simulink model "r2_b16a4x64f"  (R2012b)
(part 3 of 227)

  latch0/6(feng_chk_err_reg) -> status0/6(out_feng_chk_err)
  latch0/14(pack_err_reg) -> status0/14(out_pack_err)
  latch0/10(rx_bad_pkt_reg) -> status0/10(out_rx_bad_pkt)
  latch0/7(adc_over_reg) -> status0/7(out_adc_over)
  latch0/9(vacc_err_reg) -> status0/9(out_vacc_err)
  latch0/4(fft_err_reg) -> status0/4(out_fft_err)
  latch0/11(rx_bad_frame_reg) -> status0/11(out_rx_bad_frame)
  latch0/5(feng_qdr_err_reg) -> status0/5(out_feng_qdr_err)
  latch0/8(noise_diode_en_reg) -> status0/8(out_noise_diode_en)
  latch0/13(xeng_bad_dat_reg) -> status0/13(out_xeng_bad_dat)
  latch0/17(data_bad) -> [data_in_bad0]
  latch0/18(error) -> [err0]
  [gbe_up0] -> Inverter5/1
  [clr_status] -> latch0/1(reset)
  [pack_err0] -> latch0/15(pack_err)
  [pre_rx_dest_err0] -> latch0/3(rx_dest_err)
  [pre_feng_rx_err0] -> latch0/4(feng_rx_err)
  [pre_ndiode_en0] -> latch0/9(noise_diode_en)
  [pre_adc_err0] -> latch0/8(adc_over)
  [vacc_err0] -> latch0/10(vacc_err)
  [pre_spead_err0] -> latch0/11(rx_bad_pkt)
  [pre_feng_chk_err0] -> latch0/7(feng_chk_err)
  [gbe_rx_bad0] -> latch0/12(rx_bad_frame)
  [pre_feng_qdr_err0] -> latch0/6(feng_qdr_err)
  [gbe_tx_over0] -> latch0/13(tx_over)
  [pre_fft_err0] -> latch0/5(fft_err)
  [reord_recverr0] -> latch0/14(xeng_bad_dat)
  Inverter5/1 -> latch0/2(gbe_down)
  Inverter/1 -> latch0/16(rx)
  [accumulating0] -> latch0/17(tx)
  [reord_recverr0] -> Inverter/1
  [gbe_up1] -> Inverter7/1
  [clr_status] -> latch3/1(reset)
  [pack_err3] -> latch3/15(pack_err)
  [pre_rx_dest_err3] -> latch3/3(rx_dest_err)
  [pre_feng_rx_err3] -> latch3/4(feng_rx_err)
  [pre_ndiode_en3] -> latch3/9(noise_diode_en)
  [pre_adc_err3] -> latch3/8(adc_over)
  [vacc_err3] -> latch3/10(vacc_err)
  [pre_spead_err3] -> latch3/11(rx_bad_pkt)
  [pre_feng_chk_err3] -> latch3/7(feng_chk_err)
  [gbe_rx_bad1] -> latch3/12(rx_bad_frame)
  [pre_feng_qdr_err3] -> latch3/6(feng_qdr_err)
  [gbe_tx_over1] -> latch3/13(tx_over)
  [pre_fft_err3] -> latch3/5(fft_err)
  [reord_recverr3] -> latch3/14(xeng_bad_dat)
  Inverter7/1 -> latch3/2(gbe_down)
  Inverter6/1 -> latch3/16(rx)
  [accumulating3] -> latch3/17(tx)
  [reord_recverr3] -> Inverter6/1
  vacc_monitor7/1(pkt_cnt) -> packcnt_out3/1(out_reg)
  vacc_monitor7/2(error_cnt) -> packerr_3/1(out_reg)
  [cnt_rst] -> vacc_monitor7/1(cnt_rst)
  [pack_txeof3] -> vacc_monitor7/2(eof)
  [pack_err3] -> vacc_monitor7/3(error)
  [vacc_ld_stat3] -> Delay5/1(d)
  [err_output_of3] -> vacc_monitor11/5(outof)
  [err_parity3] -> vacc_monitor11/6(parity)
  [err_rst3] -> vacc_monitor11/4(rst)
  [err_input_of3] -> vacc_monitor11/3(inof)
  [err_calfail3] -> vacc_monitor11/2(cal)
  vacc_monitor11/1(cal_cnt) -> vacc_errors3/1(out_calfail)
  vacc_monitor11/2(inof_cnt) -> vacc_errors3/2(out_inputof)
  vacc_monitor11/3(rst_cnt) -> vacc_errors3/3(out_rst)
  vacc_monitor11/4(outof_cnt) -> vacc_errors3/4(out_outputof)
  vacc_monitor11/5(parity_cnt) -> vacc_errors3/5(out_parity)
  [vacc_err_flags3] -> bus_expand4/1(bus_in)
  miss_cnt3/3(recv_ctr) -> reordcnt_recv3/1(out_reg)
  miss_cnt3/1(spectr_cnt) -> reordcnt_spec3/1(out_reg)
  miss_cnt3/2(last_missed_ant) -> reord_missant3/1(out_reg)
  miss_cnt3/4(recv_errctr) -> reorderr_recv3/1(out_reg)
  miss_cnt3/5(timeout_errctr) -> reorderr_timeout3/1(out_reg)
  miss_cnt3/6(pktdisc_errctr) -> reorderr_disc3/1(out_reg)
  [flags_error0] -> Logical/1
  [flags_error1] -> Logical/2
  [flags_error2] -> Logical/3
  [flags_error3] -> Logical/4
  [flags_warning0] -> Logical1/1
  [flags_warning1] -> Logical1/2
  [flags_warning2] -> Logical1/3
  [flags_warning3] -> Logical1/4
  Logical/1 -> Slice/1
  Logical1/1 -> Slice1/1
  [cnt_rst] -> Delay3/2, Delay/2
  Delay/1 -> status/1(out_error)
  Delay3/1 -> status/2(out_warning)
  Slice/1 -> Delay/3, Delay/1
  Slice1/1 -> Delay3/3, Delay3/1
  Delay4/1(q) -> bus_expand5/1(bus_in)
  gapsize/1(in_gap_size) -> Register/1, Relational/2, Delay1/1
  Delay1/1 -> Relational/1
  Relational/1 -> Register/2
  Register/1 -> pipeline24/1(d), pipeline23/1(d), pipeline14/1(d), pipeline10/1(d)
  Delay5/1(q) -> bus_expand8/1(bus_in)
  [pack_ready0] -> vacc_monitor1/3(ready)
  [pack_txeof0] -> vacc_monitor1/4(eof)
  vacc_monitor1/2(ready_cnt) -> vaccout0/1(out_ready_cnt)
  vacc_monitor1/1(acc_cnt) -> vacccnt0/1(out_reg)
  vacc_monitor1/4(error_cnt) -> vaccerr0/1(out_reg)
  vacc_monitor1/3(eof_cnt) -> vaccout0/2(out_eof_cnt)
  vacc_monitor10/2(ready_cnt) -> vaccout1/1(out_ready_cnt)
  vacc_monitor10/1(acc_cnt) -> vacccnt1/1(out_reg)
  vacc_monitor10/4(error_cnt) -> vaccerr1/1(out_reg)
  vacc_monitor10/3(eof_cnt) -> vaccout1/2(out_eof_cnt)
  [vacc_err1] -> vacc_monitor10/5(error)
  [pack_txeof1] -> vacc_monitor10/4(eof)
  [pack_ready1] -> vacc_monitor10/3(ready)
  [vacc_newacc1] -> vacc_monitor10/2(new_acc)
  [cnt_rst] -> vacc_monitor10/1(cnt_rst), vacc_monitor9/1(cnt_rst)
  bus_expand7/1(msb_out2) -> vacc_ld_status2/1(out_armcnt)
  bus_expand7/2(lsb_out1) -> vacc_ld_status2/2(out_ldcnt)
  vacc_monitor4/1(acc_cnt) -> vacccnt2/1(out_reg)
  Delay39/1(q) -> bus_expand7/1(bus_in)
  [vacc_err2] -> vacc_monitor4/5(error)
  [pack_ready2] -> vacc_monitor4/3(ready)
  [pack_txeof2] -> vacc_monitor4/4(eof)
  [vacc_newacc2] -> vacc_monitor4/2(new_acc)
  bus_expand8/1(msb_out2) -> vacc_ld_status3/1(out_armcnt)
  bus_expand8/2(lsb_out1) -> vacc_ld_status3/2(out_ldcnt)
  vacc_monitor12/2(ready_cnt) -> vaccout3/1(out_ready_cnt)
  vacc_monitor12/1(acc_cnt) -> vacccnt3/1(out_reg)
  vacc_monitor12/4(error_cnt) -> vaccerr3/1(out_reg)
  vacc_monitor12/3(eof_cnt) -> vaccout3/2(out_eof_cnt)
  [pack_ready2] -> vacc_monitor12/3(ready)
  [pack_txeof2] -> vacc_monitor12/4(eof)
  [vacc_err3] -> vacc_monitor12/5(error)
  [cnt_rst] -> vacc_monitor12/1(cnt_rst), vacc_monitor11/1(cnt_rst)
  [vacc_newacc3] -> vacc_monitor12/2(new_acc)
  vacc_monitor4/4(error_cnt) -> vaccerr2/1(out_reg)
  vacc_monitor4/3(eof_cnt) -> vaccout2/2(out_eof_cnt)
  vacc_monitor4/2(ready_cnt) -> vaccout2/1(out_ready_cnt)
  [flush0] -> latch0/18(flush)
  latch0/19(flush_reg) -> status0/17(out_flushed)
  [flush0] -> latch1/18(flush)
  latch1/15(rx_reg) -> status1/15(out_rxing_data)
  latch1/6(feng_chk_err_reg) -> status1/6(out_feng_chk_err)
  latch1/1(gbe_down_reg) -> status1/1(out_gbe_down)
  latch1/12(tx_over_reg) -> status1/12(out_tx_over)
  latch1/13(xeng_bad_dat_reg) -> status1/13(out_xeng_bad_dat)
  latch1/10(rx_bad_pkt_reg) -> status1/10(out_rx_bad_pkt)
  latch1/9(vacc_err_reg) -> status1/9(out_vacc_err)
  latch1/2(rx_dest_err_reg) -> status1/2(out_rx_dest_err)
  latch1/3(feng_rx_err_reg) -> status1/3(out_feng_rx_err)
  latch1/11(rx_bad_frame_reg) -> status1/11(out_rx_bad_frame)
  latch1/7(adc_over_reg) -> status1/7(out_adc_over)
  latch1/5(feng_qdr_err_reg) -> status1/5(out_feng_qdr_err)
  latch1/14(pack_err_reg) -> status1/14(out_pack_err)
  latch1/16(tx_reg) -> status1/16(out_txing_data)
  latch1/8(noise_diode_en_reg) -> status1/8(out_noise_diode_en)
  latch1/4(fft_err_reg) -> status1/4(out_fft_err)
  latch1/17(data_bad) -> [data_in_bad1]
  latch1/18(error) -> [err1]
  latch1/19(flush_reg) -> status1/17(out_flushed)
  [flush1] -> latch2/18(flush)
  [flush1] -> latch3/18(flush)
  latch2/14(pack_err_reg) -> status2/14(out_pack_err)
  latch2/7(adc_over_reg) -> status2/7(out_adc_over)
  latch2/10(rx_bad_pkt_reg) -> status2/10(out_rx_bad_pkt)
  latch2/1(gbe_down_reg) -> status2/1(out_gbe_down)
  latch2/16(tx_reg) -> status2/16(out_txing_data)
  latch2/6(feng_chk_err_reg) -> status2/6(out_feng_chk_err)
  latch2/12(tx_over_reg) -> status2/12(out_tx_over)
  latch2/11(rx_bad_frame_reg) -> status2/11(out_rx_bad_frame)
  latch2/2(rx_dest_err_reg) -> status2/2(out_rx_dest_err)
  latch2/8(noise_diode_en_reg) -> status2/8(out_noise_diode_en)
  latch2/3(feng_rx_err_reg) -> status2/3(out_feng_rx_err)
  latch2/15(rx_reg) -> status2/15(out_rxing_data)
  latch2/5(feng_qdr_err_reg) -> status2/5(out_feng_qdr_err)
  latch2/4(fft_err_reg) -> status2/4(out_fft_err)
  latch2/9(vacc_err_reg) -> status2/9(out_vacc_err)
  latch2/13(xeng_bad_dat_reg) -> status2/13(out_xeng_bad_dat)
  latch2/17(data_bad) -> [data_in_bad2]
  latch2/18(error) -> [err2]
  latch2/19(flush_reg) -> status2/17(out_flushed)
  latch3/6(feng_chk_err_reg) -> status3/6(out_feng_chk_err)
  latch3/1(gbe_down_reg) -> status3/1(out_gbe_down)
  latch3/12(tx_over_reg) -> status3/12(out_tx_over)
  latch3/13(xeng_bad_dat_reg) -> status3/13(out_xeng_bad_dat)
  latch3/15(rx_reg) -> status3/15(out_rxing_data)
  latch3/7(adc_over_reg) -> status3/7(out_adc_over)
  latch3/8(noise_diode_en_reg) -> status3/8(out_noise_diode_en)
  latch3/11(rx_bad_frame_reg) -> status3/11(out_rx_bad_frame)
  latch3/16(tx_reg) -> status3/16(out_txing_data)
  latch3/10(rx_bad_pkt_reg) -> status3/10(out_rx_bad_pkt)
  latch3/9(vacc_err_reg) -> status3/9(out_vacc_err)
  latch3/3(feng_rx_err_reg) -> status3/3(out_feng_rx_err)
  latch3/14(pack_err_reg) -> status3/14(out_pack_err)
  latch3/4(fft_err_reg) -> status3/4(out_fft_err)
  latch3/5(feng_qdr_err_reg) -> status3/5(out_feng_qdr_err)
  latch3/2(rx_dest_err_reg) -> status3/2(out_rx_dest_err)
  latch3/17(data_bad) -> [data_in_bad3]
  latch3/19(flush_reg) -> status3/17(out_flushed)
  latch3/18(error) -> [err3]
  bus_expand2/1(msb_out5) -> [err_parity0]
  bus_expand2/2(out4) -> [err_output_of0]
  bus_expand2/3(out3) -> [err_rst0]
  bus_expand2/4(out2) -> [err_input_of0]
  bus_expand2/5(lsb_out1) -> [err_calfail0]
  bus_expand1/1(msb_out5) -> [err_parity1]
  bus_expand1/2(out4) -> [err_output_of1]
  bus_expand1/3(out3) -> [err_rst1]
  bus_expand1/4(out2) -> [err_input_of1]
  bus_expand1/5(lsb_out1) -> [err_calfail1]
  bus_expand9/1(msb_out5) -> [err_parity2]
  bus_expand9/2(out4) -> [err_output_of2]
  bus_expand9/3(out3) -> [err_rst2]
  bus_expand9/4(out2) -> [err_input_of2]
  bus_expand9/5(lsb_out1) -> [err_calfail2]
  bus_expand4/1(msb_out5) -> [err_parity3]
  bus_expand4/2(out4) -> [err_output_of3]
  bus_expand4/3(out3) -> [err_rst3]
  bus_expand4/4(out2) -> [err_input_of3]
  bus_expand4/5(lsb_out1) -> [err_calfail3]
  [pre_rx_dest_err0] -> Subsystem5/5(dest_err)
  Subsystem5/3(desterr_cnt) -> dest_err_cnt0/1(out_reg)
  [spead_error1] -> Subsystem2/4(flag)
  [spead_eof1] -> Subsystem2/3(eof)
  [spead_valid1] -> Subsystem2/2(we)
  Subsystem2/1(rx_cnt) -> rx_cnt1/1(out_reg)
  Subsystem2/2(err_cnt) -> rx_err_cnt1/1(out_reg)
  Subsystem2/3(desterr_cnt) -> dest_err_cnt1/1(out_reg)
  [pre_rx_dest_err1] -> Subsystem2/5(dest_err)
  Constant4/1 -> gbe2/7(rx_ack)
  Constant5/1 -> gbe2/8(rx_overrun_ack)
  Constant6/1 -> gbe3/7(rx_ack)
  Constant3/1 -> gbe3/8(rx_overrun_ack)
  [gbe_debug_rst] -> gbe2/9(debug_rst)
  [gbe_debug_rst] -> gbe3/9(debug_rst)
  [gbe_rst] -> gbe2/1(rst)
  [gbe_txd2] -> gbe2/2(tx_data)
  [gbe_txvld2] -> gbe2/3(tx_valid)
  [gbe_txeof2] -> gbe2/6(tx_end_of_frame)
  [gbe_rst] -> gbe3/1(rst)
  [gbe_txd3] -> gbe3/2(tx_data)
  [gbe_txvld3] -> gbe3/3(tx_valid)
  [gbe_txeof3] -> gbe3/6(tx_end_of_frame)
  Constant7/1 -> [gbe_txd2]
  Constant10/1 -> [gbe_txvld2]
  Constant11/1 -> [gbe_txeof2]
  Constant15/1 -> [gbe_txd3]
  Constant12/1 -> [gbe_txvld3]
  Constant14/1 -> [gbe_txeof3]
  [gbe_rxvld2] -> Delay41/1(d)
  [gbe_rxdata2] -> Delay40/1(d)
  [gbe_rxeof2] -> Delay42/1(d)
  Delay40/1(q) -> spead_unpack2/1(pkt_data)
  Delay41/1(q) -> spead_unpack2/2(pkt_valid)
  Delay42/1(q) -> spead_unpack2/3(pkt_eof)
  [gbe_rxvld3] -> Delay44/1(d)
  [gbe_rxdata3] -> Delay43/1(d)
  [gbe_rxeof3] -> Delay45/1(d)
  Delay43/1(q) -> spead_unpack3/1(pkt_data)
  Delay44/1(q) -> spead_unpack3/2(pkt_valid)
  Delay45/1(q) -> spead_unpack3/3(pkt_eof)
  [cnt_rst] -> Subsystem1/1(rst)
  [spead_error2] -> Subsystem1/4(flag)
  [spead_eof2] -> Subsystem1/3(eof)
  [spead_valid2] -> Subsystem1/2(we)
  Subsystem1/1(rx_cnt) -> rx_cnt2/1(out_reg)
  Subsystem1/2(err_cnt) -> rx_err_cnt2/1(out_reg)
  Subsystem1/3(desterr_cnt) -> dest_err_cnt2/1(out_reg)
  [pre_rx_dest_err2] -> Subsystem1/5(dest_err)
  [cnt_rst] -> Subsystem3/1(rst)
  [spead_error3] -> Subsystem3/4(flag)
  [spead_eof3] -> Subsystem3/3(eof)
  [spead_valid3] -> Subsystem3/2(we)
  Subsystem3/1(rx_cnt) -> rx_cnt3/1(out_reg)
  Subsystem3/2(err_cnt) -> rx_err_cnt3/1(out_reg)
  Subsystem3/3(desterr_cnt) -> dest_err_cnt3/1(out_reg)
  [pre_rx_dest_err3] -> Subsystem3/5(dest_err)
  bf_config/1(in_data_id) -> pipeline26/1(d)
  bf_config/2(in_time_id) -> pipeline27/1(d)
  bf_control/2(in_stream) -> pipeline29/1(d)
  bf_control/3(in_antenna) -> pipeline30/1(d)
  bf_control/1(in_beng) -> pipeline28/1(d)
  pipeline26/1(q) -> [bf_data_id]
  pipeline27/1(q) -> [bf_time_id]
  pipeline28/1(q) -> [bf_beng]
  pipeline29/1(q) -> [bf_stream]
  pipeline30/1(q) -> [bf_antenna]
  pipeline53/1(q) -> [bf_value_filt]
  pipeline54/1(q) -> [bf_value_dupl]
  pipeline55/1(q) -> [bf_value_bw]
  pipeline56/1(q) -> [bf_value_quant]
  bf_value_in0/1(in_dupl) -> pipeline54/1(d)
  bf_value_in1/1(in_quant) -> pipeline56/1(d)
  bf_value_in1/2(in_filt) -> pipeline53/1(d)
  bf_value_ctrl/1(in_dupl) -> pipeline32/1(d)
  bf_value_ctrl/3(in_quant) -> pipeline34/1(d)
  pipeline32/1(q) -> edge_detect6/1
  pipeline33/1(q) -> edge_detect7/1
  pipeline34/1(q) -> edge_detect8/1
  pipeline57/1(q) -> edge_detect9/1
  bf_value_ctrl/2(in_bw) -> pipeline33/1(d)
  bf_value_ctrl/4(in_filt) -> pipeline57/1(d)
  bf_value_in0/2(in_bw) -> pipeline55/1(d)
  [bfout_valbw0] -> Delay27/1(d)
  [bfout_valquant0] -> Delay30/1(d)
  [bfout_valfilt0] -> Delay31/1(d)
  [bfout_valbw1] -> Delay26/1(d)
  [bfout_valbw2] -> Delay28/1(d)
  [bfout_valbw3] -> Delay32/1(d)
  [bfout_valquant1] -> Delay33/1(d)
  [bfout_valquant2] -> Delay35/1(d)
  [bfout_valquant3] -> Delay36/1(d)
  [bfout_valfilt1] -> Delay37/1(d)
  [bfout_valfilt2] -> Delay38/1(d)
  [bfout_valfilt3] -> Delay46/1(d)
  Delay27/1(q) -> bf_valout_bw0/1(out_bw0)
  Delay26/1(q) -> bf_valout_bw0/2(out_bw1)
  Delay32/1(q) -> bf_valout_bw1/2(out_bw3)
  Delay28/1(q) -> bf_valout_bw1/1(out_bw2)
  Delay30/1(q) -> bf_valout_quant0/1(out_quant0)
  Delay33/1(q) -> bf_valout_quant0/2(out_quant1)
  Delay36/1(q) -> bf_valout_quant1/2(out_quant3)
  Delay35/1(q) -> bf_valout_quant1/1(out_quant2)
  Delay37/1(q) -> bf_valout_filt/2(out_filt1)
  Delay38/1(q) -> bf_valout_filt/3(out_filt2)
  Delay46/1(q) -> bf_valout_filt/4(out_filt3)
  Delay31/1(q) -> bf_valout_filt/1(out_filt0)
  edge_detect6/1 -> [bf_valctrl_dupl]
  edge_detect7/1 -> [bf_valctrl_bw]
  edge_detect8/1 -> [bf_valctrl_quant]
  edge_detect9/1 -> [bf_valctrl_filt]
  Concat5/1 -> gbe_mux_bus0/1(di)
  [pack_txd1] -> Concat5/2
  [pack_txd0] -> Concat5/1
  Concat6/1 -> gbe_mux_bus0/2(validi)
  Concat7/1 -> gbe_mux_bus0/3(eofi)
  gbe_mux_bus0/5(start) -> Delay12/1, bus_expand/1(bus_in)
  Concat9/1 -> gbe_mux_bus0/4(drdy)
  Constant26/1 -> gbe_mux_bus0/5(transmit)
  gbe_mux_bus0/2(do) -> Delay13/1
  gbe_mux_bus0/3(valido) -> Delay14/1
  gbe_mux_bus0/4(eofo) -> Delay15/1
  gbe_mux_bus0/6(flush) -> [flush0]
  [bf0s_d0] -> Concat5/3
  [bf1s_d0] -> Concat5/4
  [pack_txvld0] -> Concat6/1
  [pack_txvld1] -> Concat6/2
  [bf0s_en0] -> Concat6/3
  [bf1s_en0] -> Concat6/4
  [bf0s_eof0] -> Concat7/3
  [bf1s_eof0] -> Concat7/4
  [pack_txeof0] -> Concat7/1
  [pack_txeof1] -> Concat7/2
  [bf0s_pkt_ready0] -> Concat9/3
  [bf1s_pkt_ready0] -> Concat9/4
  [pack_ready1] -> Concat9/2
  [pack_ready0] -> Concat9/1
  [bf0s_d1] -> Concat5/5
  [bf1s_d1] -> Concat5/6
  [bf0s_en1] -> Concat6/5
  [bf1s_en1] -> Concat6/6
  [bf0s_eof1] -> Concat7/5
  [bf1s_eof1] -> Concat7/6
  [bf0s_pkt_ready1] -> Concat9/5
  [bf1s_pkt_ready1] -> Concat9/6
  bus_expand/1(msb_out6) -> [go0]
  bus_expand/2(out5) -> [go1]
  bus_expand/3(out4) -> [bf0_tx_pkt0]
  bus_expand/4(out3) -> [bf1_tx_pkt0]
  bus_expand/5(out2) -> [bf0_tx_pkt1]
  bus_expand/6(lsb_out1) -> [bf1_tx_pkt1]
  Concat1/1 -> gbe_mux_bus/1(di)
  Concat2/1 -> gbe_mux_bus/2(validi)
  Concat3/1 -> gbe_mux_bus/3(eofi)
  gbe_mux_bus/5(start) -> bus_expand3/1(bus_in)
  Concat4/1 -> gbe_mux_bus/4(drdy)
  Constant1/1 -> gbe_mux_bus/5(transmit)
  gbe_mux_bus/2(do) -> Delay24/1
  gbe_mux_bus/4(eofo) -> Delay22/1
  gbe_mux_bus/6(flush) -> [flush1]
  gbe_mux_bus/3(valido) -> Delay23/1
  [pack_txd2] -> Concat1/1
  [pack_txd3] -> Concat1/2
  [pack_txvld2] -> Concat2/1
  [pack_txvld3] -> Concat2/2
  [pack_txeof2] -> Concat3/1
  [pack_txeof3] -> Concat3/2
  [pack_ready2] -> Concat4/1
  [pack_ready3] -> Concat4/2
  bus_expand3/1(msb_out6) -> [go2]
  bus_expand3/2(out5) -> [go3]
  [bf0s_d2] -> Concat1/3
  [bf1s_d2] -> Concat1/4
  [bf0s_d3] -> Concat1/5
  [bf1s_d3] -> Concat1/6
  [bf0s_en2] -> Concat2/3
  [bf1s_en2] -> Concat2/4
  [bf0s_en3] -> Concat2/5
  [bf1s_en3] -> Concat2/6
  [bf0s_eof2] -> Concat3/3
  [bf1s_eof2] -> Concat3/4
  [bf0s_eof3] -> Concat3/5
  [bf1s_eof3] -> Concat3/6
  [bf0s_pkt_ready2] -> Concat4/3
  [bf1s_pkt_ready2] -> Concat4/4
  [bf0s_pkt_ready3] -> Concat4/5
  [bf1s_pkt_ready3] -> Concat4/6
  bus_expand3/3(out4) -> [bf0_tx_pkt2]
  bus_expand3/4(out3) -> [bf1_tx_pkt2]
  bus_expand3/5(out2) -> [bf0_tx_pkt3]
  bus_expand3/6(lsb_out1) -> [bf1_tx_pkt3]
  Delay13/1 -> [gbe_txd0]
  Delay14/1 -> [gbe_txvld0]
  Delay15/1 -> [gbe_txeof0]
  gbe_mux_bus0/1(input) -> Mux2/1, Delay11/1, Mux1/1
  AddSub7/1 -> Mux1/5
  AddSub4/1 -> Mux1/4
  [bf0_txport] -> Mux2/6, Mux2/4
  [bf1_txport] -> Mux2/7, Mux2/5
  [gbe_txport] -> Mux2/3, Mux2/2
  Mux2/1 -> [gbe_txport0]
  Delay22/1 -> [gbe_txeof1]
  Delay23/1 -> [gbe_txvld1]
  Delay24/1 -> [gbe_txd1]
  gbe_mux_bus/1(input) -> Mux3/1, Mux4/1
  AddSub13/1 -> Mux3/5
  AddSub10/1 -> Mux3/4
  [bf0_txport] -> Mux4/4, Mux4/6
  [bf1_txport] -> Mux4/7, Mux4/5
  [gbe_txport] -> Mux4/2, Mux4/3
  Mux3/1 -> [gbe_txip1]
  Mux4/1 -> [gbe_txport1]
  Delay11/1 -> [gbe_ipsel0]
  Delay12/1 -> [gbe_txstart0]
  Mux1/1 -> [gbe_txip0]
  Constant18/1 -> gbe3/4(tx_dest_ip)
  Constant19/1 -> gbe3/5(tx_dest_port)
  Constant16/1 -> gbe2/4(tx_dest_ip)
  Constant17/1 -> gbe2/5(tx_dest_port)
  pipeline59/1(q) -> [bf_tvgsel]
  bf_config/3(in_tvg_sel) -> pipeline59/1(d)
  pipeline60/1(q) -> [bf_snap_arm]
  pipeline61/1(q) -> [bf_snap_trig]
  bf_config/4(in_snap_arm) -> pipeline60/1(d)
  bf_config/5(in_snap_trig) -> pipeline61/1(d)
  [bfout_sync0] -> Delay53/1(d)
  [bf_snap_arm] -> Logical4/1
  Delay53/1(q) -> Logical4/2
  Logical4/1 -> Logical5/1
  [bf_snap_trig] -> edge_detect10/1
  edge_detect10/1 -> Logical5/2
  Logical5/1 -> bfsnap_out/6(trig)
  [bfout_sync0] -> Delay54/1(d)
  [bfout_den0] -> slice1/1
  Delay56/1(q) -> bfsnap_out/3(in_d32)
  [bfout_d0] -> Delay56/1(d)
  Delay57/1(q) -> slice5/1
  [bfout_time0] -> Delay57/1(d)
  Delay54/1(q) -> bfsnap_out/1(in_sync)
  Delay55/1(q) -> bfsnap_out/2(in_en), bfsnap_out/5(we)
  slice5/1 -> bfsnap_out/4(in_time27)
  slice1/1 -> Delay55/1(d)
  vacctvg_control/1(in_sync_sel) -> pipeline65/1(d)
  vacctvg_control/2(in_valid_sel) -> pipeline62/1(d)
  vacctvg_control/3(in_data_sel) -> pipeline66/1(d)
  vacctvg_control/4(in_reset) -> pipeline64/1(d)
  vacctvg_control/5(in_ctr_en) -> pipeline69/1(d)
  vacctvg_control/6(in_vector_en) -> pipeline67/1(d)
  vacctvg_control/7(in_pulse_en) -> pipeline70/1(d)
  pipeline65/1(q) -> [vacctvg_sync_sel]
  pipeline62/1(q) -> [vacctvg_valid_sel]
  pipeline64/1(q) -> [vacctvg_reset]
  pipeline66/1(q) -> [vacctvg_data_sel]
  pipeline67/1(q) -> [vacctvg_vector_en]
  pipeline69/1(q) -> [vacctvg_ctr_en]
  pipeline70/1(q) -> [vacctvg_pulse_en]
  pipeline68/1(q) -> [vacctvg_vbs_rst0]
  vacctvg_control/8(in_vbs_rst0) -> pipeline68/1(d)
  pipeline71/1(q) -> [vacctvg_vbs_rst1]
  pipeline63/1(q) -> [vacctvg_vbs_rst2]
  pipeline72/1(q) -> [vacctvg_vbs_rst3]
  vacctvg_control/9(in_vbs_rst1) -> pipeline71/1(d)
  vacctvg_control/10(in_vbs_rst2) -> pipeline63/1(d)
  vacctvg_control/11(in_vbs_rst3) -> pipeline72/1(d)
  bf1_config/2(in_beam_id) -> pipeline58/1(d)
  bf1_config/1(in_rst) -> pipeline45/1(d)
  pipeline45/1(q) -> [bf1_rst]
  pipeline58/1(q) -> Convert1/1
  bf1_config/3(in_port) -> pipeline43/1(d)
  pipeline43/1(q) -> [bf1_txport]
  pipeline44/1(q) -> [bf1_txen]
  bf1_config/4(in_txen) -> pipeline44/1(d)
  Convert1/1 -> [bf1_id]
  pipeline37/1(q) -> [bf1_n_partitions]
  bf0_config/2(in_beam_id) -> pipeline50/1(d)
  bf0_config/1(in_rst) -> pipeline38/1(d)
  pipeline38/1(q) -> [bf0_rst]
  pipeline50/1(q) -> Convert2/1
  bf0_config/3(in_port) -> pipeline35/1(d)
  pipeline35/1(q) -> [bf0_txport]
  pipeline36/1(q) -> [bf0_txen]
  bf0_config/4(in_txen) -> pipeline36/1(d)
  Convert2/1 -> [bf0_id]
  bf0_num_parts/1(in_n_partitions) -> pipeline31/1(d)
  pipeline31/1(q) -> [bf0_n_partitions]
  bf0_partitions/1(in_partition0_offset) -> pipeline39/1(d)
  bf0_partitions/2(in_partition1_offset) -> pipeline40/1(d)
  bf0_partitions/3(in_partition2_offset) -> pipeline41/1(d)
  bf0_partitions/4(in_partition3_offset) -> pipeline42/1(d)
  bf1_partitions/1(in_partition0_offset) -> pipeline46/1(d)
  bf1_partitions/2(in_partition1_offset) -> pipeline47/1(d)
  bf1_partitions/3(in_partition2_offset) -> pipeline48/1(d)
  bf1_partitions/4(in_partition3_offset) -> pipeline49/1(d)
  pipeline39/1(q) -> [bf0_partition_offset0]
  pipeline40/1(q) -> [bf0_partition_offset1]
  pipeline41/1(q) -> [bf0_partition_offset2]
  pipeline42/1(q) -> [bf0_partition_offset3]
  pipeline46/1(q) -> [bf1_partition_offset0]
  pipeline47/1(q) -> [bf1_partition_offset1]
  pipeline48/1(q) -> [bf1_partition_offset2]
  pipeline49/1(q) -> [bf1_partition_offset3]
  bf0_ip/1(in_ip) -> pipeline51/1(d)
  pipeline51/1(q) -> [bf0_txip]
  bf1_ip/1(in_ip) -> pipeline52/1(d)
  pipeline52/1(q) -> [bf1_txip]
  [cnt_rst] -> Subsystem/1(rst)
  [bf0s_eof0] -> Subsystem/2(of0)
  Subsystem/1(Out1) -> bf0_out_count/1(out_count0)
  [bf0s_eof2] -> Subsystem/4(of2)
  [bf0s_eof1] -> Subsystem/3(of1)
  [bf0s_eof3] -> Subsystem/5(of3)
  Subsystem/2(Out2) -> bf0_out_count/2(out_count1)
  Subsystem/3(Out3) -> bf0_out_count/3(out_count2)
  Subsystem/4(Out4) -> bf0_out_count/4(out_count3)
  [cnt_rst] -> Subsystem4/1(rst)
  [bf0s_of0] -> Subsystem4/2(of0)
  Subsystem4/1(Out1) -> bf0_of_count/1(out_count0)
  [bf0s_of2] -> Subsystem4/4(of2)
  [bf0s_of1] -> Subsystem4/3(of1)
  [bf0s_of3] -> Subsystem4/5(of3)
  Subsystem4/2(Out2) -> bf0_of_count/2(out_count1)
  Subsystem4/3(Out3) -> bf0_of_count/3(out_count2)
  Subsystem4/4(Out4) -> bf0_of_count/4(out_count3)
  [cnt_rst] -> Subsystem6/1(rst)
  [bf1s_eof0] -> Subsystem6/2(of0)
  Subsystem6/1(Out1) -> bf1_out_count/1(out_count0)
  [bf1s_eof2] -> Subsystem6/4(of2)
  [bf1s_eof1] -> Subsystem6/3(of1)
  [bf1s_eof3] -> Subsystem6/5(of3)
  Subsystem6/2(Out2) -> bf1_out_count/2(out_count1)
  Subsystem6/3(Out3) -> bf1_out_count/3(out_count2)
  Subsystem6/4(Out4) -> bf1_out_count/4(out_count3)
  [cnt_rst] -> Subsystem7/1(rst)
  [bf1s_of0] -> Subsystem7/2(of0)
  Subsystem7/1(Out1) -> bf1_of_count/1(out_count0)
  [bf1s_of2] -> Subsystem7/4(of2)
  [bf1s_of1] -> Subsystem7/3(of1)
  [bf1s_of3] -> Subsystem7/5(of3)
  Subsystem7/3(Out3) -> bf1_of_count/3(out_count2)
  Subsystem7/4(Out4) -> bf1_of_count/4(out_count3)
  Subsystem7/2(Out2) -> bf1_of_count/2(out_count1)
  bf1_num_parts/1(in_n_partitions) -> pipeline37/1(d)
  gbe0/1(led_up) -> [gbe_up0]
  gbe0/3(led_tx) -> Terminator1/1
  gbe0/2(led_rx) -> Terminator7/1
  gbe0/4(tx_afull) -> Terminator13/1
  gbe0/5(tx_overflow) -> [gbe_tx_over0]
  gbe0/6(rx_data) -> [gbe_rxdata0]
  gbe0/7(rx_valid) -> [gbe_rxvld0]
  gbe0/8(rx_source_ip) -> Terminator14/1
  gbe0/9(rx_source_port) -> Terminator15/1
  gbe0/10(rx_end_of_frame) -> [gbe_rxeof0]
  gbe0/11(rx_bad_frame) -> [gbe_rx_bad0]
  gbe0/12(rx_overrun) -> Terminator35/1
  gbe0/13(rx_dest_ip) -> Terminator36/1
  gbe0/14(rx_dest_port) -> Terminator45/1
  gbe1/1(led_up) -> [gbe_up1]
  gbe1/2(led_rx) -> Terminator47/1
  gbe1/3(led_tx) -> Terminator38/1
  gbe1/4(tx_afull) -> Terminator46/1
  gbe1/5(tx_overflow) -> [gbe_tx_over1]
  gbe1/6(rx_data) -> [gbe_rxdata1]
  gbe1/7(rx_valid) -> [gbe_rxvld1]
  gbe1/8(rx_source_ip) -> Terminator48/1
  gbe1/9(rx_source_port) -> Terminator49/1
  gbe1/10(rx_end_of_frame) -> [gbe_rxeof1]
  gbe1/11(rx_bad_frame) -> [gbe_rx_bad1]
  gbe1/12(rx_overrun) -> Terminator50/1
  gbe1/13(rx_dest_ip) -> Terminator51/1
  gbe1/14(rx_dest_port) -> Terminator52/1
  gbe2/1(led_up) -> [gbe_up2]
  gbe2/5(tx_overflow) -> [gbe_tx_over2]
  gbe2/6(rx_data) -> [gbe_rxdata2]
  gbe2/7(rx_valid) -> [gbe_rxvld2]
  gbe2/10(rx_end_of_frame) -> [gbe_rxeof2]
  gbe2/11(rx_bad_frame) -> [gbe_rx_bad2]
  gbe3/1(led_up) -> [gbe_up3]
  gbe3/5(tx_overflow) -> [gbe_tx_over3]
  gbe3/6(rx_data) -> [gbe_rxdata3]
  gbe3/7(rx_valid) -> [gbe_rxvld3]
  gbe3/10(rx_end_of_frame) -> [gbe_rxeof3]
  gbe3/11(rx_bad_frame) -> [gbe_rx_bad3]
  gbe2/12(rx_overrun) -> Terminator6/1
  gbe2/13(rx_dest_ip) -> Terminator8/1
  gbe2/14(rx_dest_port) -> Terminator9/1
  gbe2/2(led_rx) -> Terminator10/1
  gbe2/3(led_tx) -> Terminator12/1
  gbe2/4(tx_afull) -> Terminator16/1
  gbe2/8(rx_source_ip) -> Terminator20/1
  gbe2/9(rx_source_port) -> Terminator21/1
  gbe3/12(rx_overrun) -> Terminator22/1
  gbe3/13(rx_dest_ip) -> Terminator24/1
  gbe3/14(rx_dest_port) -> Terminator25/1
  gbe3/2(led_rx) -> Terminator26/1
  gbe3/3(led_tx) -> Terminator53/1
  gbe3/4(tx_afull) -> Terminator54/1
  gbe3/8(rx_source_ip) -> Terminator55/1
  gbe3/9(rx_source_port) -> Terminator56/1
  [gbe_txip] -> AddSub6/1
  AddSub6/1 -> Mux1/2
  AddSub1/1 -> Mux1/3
  [gbe_txip] -> AddSub1/1
  [id1] -> AddSub5/2, AddSub8/2, AddSub1/2
  [gbe_txip] -> AddSub2/1
  [id2] -> AddSub13/2, AddSub10/2, AddSub2/2
  [gbe_txip] -> AddSub3/1
  [id3] -> AddSub3/2, AddSub14/2, AddSub11/2
  AddSub3/1 -> Mux3/3
  AddSub2/1 -> Mux3/2
  spead_unpack0/10(hdr5_0x1600_DIR) -> [spead_hdr1_0]
  spead_unpack0/11(hdr6_0x4101_DIR) -> [spead_hdr2_0]
  spead_unpack0/12(hdr7_0x4103_DIR) -> [spead_hdr3_0]
  spead_unpack0/13(hdr8_0x0000_DIR) -> Terminator33/1
  spead_unpack0/14(hdr9_0x0000_DIR) -> Terminator19/1
  spead_unpack0/15(hdr10_0x0000_DIR) -> Terminator4/1
  spead_unpack0/16(hdr11_0x4300) -> Terminator31/1
  spead_unpack1/2(data64) -> [spead_data1]
  spead_unpack1/3(valid64) -> [spead_valid1]
  spead_unpack1/4(eof64) -> [spead_eof1]
  spead_unpack1/5(error) -> [spead_error1]
  spead_unpack1/6(hdr_heap_id) -> Terminator17/1
  spead_unpack1/7(hdr_heap_size) -> Terminator18/1
  spead_unpack1/8(hdr_heap_offset) -> [spead_heap_offset1]
  spead_unpack1/9(hdr_pkt_len) -> Terminator32/1
  spead_unpack1/10(hdr5_0x1600_DIR) -> [spead_hdr1_1]
  spead_unpack1/11(hdr6_0x4101_DIR) -> [spead_hdr2_1]
  spead_unpack1/12(hdr7_0x4103_DIR) -> [spead_hdr3_1]
  spead_unpack1/16(hdr11_0x4300) -> Terminator42/1
  spead_unpack1/15(hdr10_0x0000_DIR) -> Terminator58/1
  spead_unpack1/14(hdr9_0x0000_DIR) -> Terminator11/1
  spead_unpack1/13(hdr8_0x0000_DIR) -> Terminator57/1
  spead_unpack2/1(pkt_start) -> Terminator34/1
  spead_unpack2/2(data64) -> [spead_data2]
  spead_unpack2/3(valid64) -> [spead_valid2]
  spead_unpack2/4(eof64) -> [spead_eof2]
  spead_unpack2/5(error) -> [spead_error2]
  spead_unpack2/6(hdr_heap_id) -> Terminator29/1
  spead_unpack2/7(hdr_heap_size) -> Terminator30/1
  spead_unpack2/8(hdr_heap_offset) -> [spead_heap_offset2]
  spead_unpack2/9(hdr_pkt_len) -> Terminator27/1
  spead_unpack2/10(hdr5_0x1600_DIR) -> [spead_hdr1_2]
  spead_unpack2/11(hdr6_0x4101_DIR) -> [spead_hdr2_2]
  spead_unpack2/12(hdr7_0x4103_DIR) -> [spead_hdr3_2]
  spead_unpack2/13(hdr8_0x0000_DIR) -> Terminator61/1
  spead_unpack2/14(hdr9_0x0000_DIR) -> Terminator60/1
  spead_unpack2/15(hdr10_0x0000_DIR) -> Terminator59/1
  spead_unpack2/16(hdr11_0x4300) -> Terminator37/1
  spead_unpack3/1(pkt_start) -> Terminator43/1
  spead_unpack3/2(data64) -> [spead_data3]
  spead_unpack3/3(valid64) -> [spead_valid3]
  spead_unpack3/4(eof64) -> [spead_eof3]
  spead_unpack3/5(error) -> [spead_error3]
  spead_unpack3/8(hdr_heap_offset) -> [spead_heap_offset3]
  spead_unpack3/6(hdr_heap_id) -> Terminator40/1
  spead_unpack3/7(hdr_heap_size) -> Terminator41/1
  spead_unpack3/9(hdr_pkt_len) -> Terminator39/1
  spead_unpack3/10(hdr5_0x1600_DIR) -> [spead_hdr1_3]
  spead_unpack3/11(hdr6_0x4101_DIR) -> [spead_hdr2_3]
  spead_unpack3/12(hdr7_0x4103_DIR) -> [spead_hdr3_3]
  spead_unpack3/13(hdr8_0x0000_DIR) -> Terminator64/1
  spead_unpack3/14(hdr9_0x0000_DIR) -> Terminator63/1
  spead_unpack3/15(hdr10_0x0000_DIR) -> Terminator62/1
  spead_unpack3/16(hdr11_0x4300) -> Terminator44/1
  [bf0_txip] -> AddSub8/1, AddSub4/1
  [id0] -> AddSub7/2, AddSub4/2, AddSub6/2
  [bf1_txip] -> AddSub5/1, AddSub7/1
  AddSub8/1 -> Mux1/6
  AddSub5/1 -> Mux1/7
  [bf0_txip] -> AddSub10/1, AddSub14/1
  [bf1_txip] -> AddSub13/1, AddSub11/1
  AddSub14/1 -> Mux3/6
  AddSub11/1 -> Mux3/7
